simulink model "AGC_script"  (R2024b)
settings: Solver=VariableStepAuto  StartTime=0.0  StopTime=7*60  RelTol=1e-3
libraries: audiomeasurements x7, dspvision x7
settings Model: Creator=Pedro  LastModifiedBy=Pedro

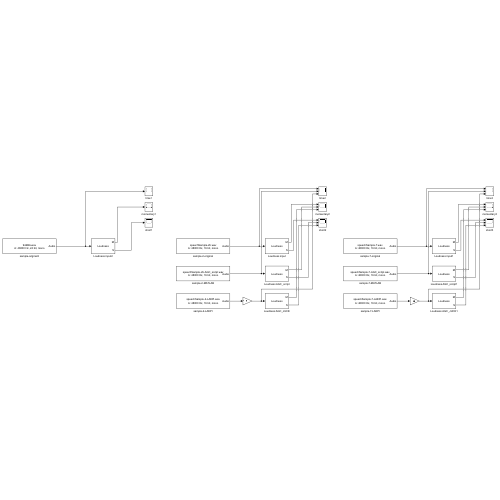
[thumbnail: Simulink's stored preview of the top-level diagram]
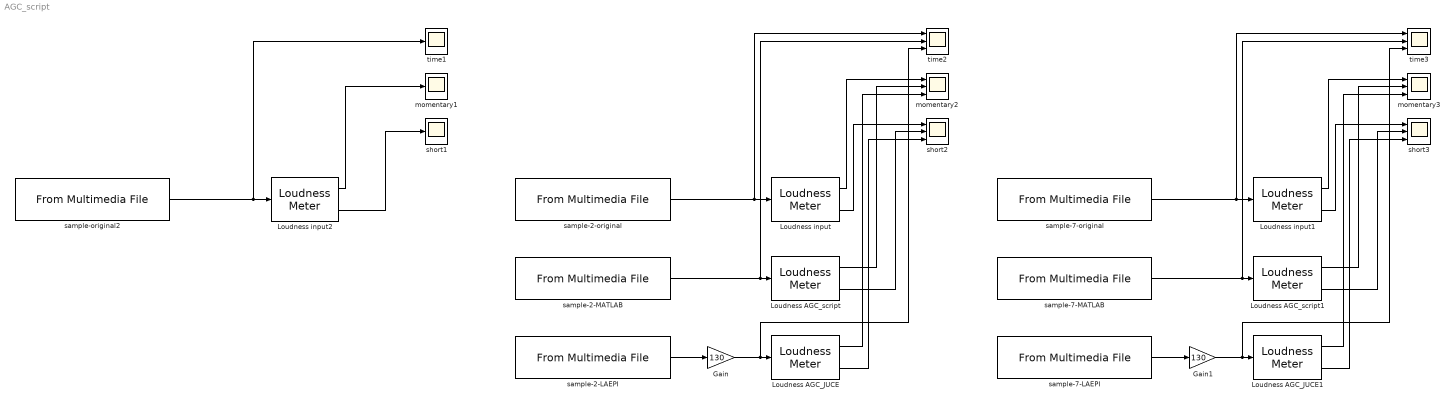
== system AGC_script ==
  Gain : Gain  Gain=130
  Gain1 : Gain  Gain=130
  Loudness AGC_JUCE : audiomeasurements/Loudness Meter  ChannelWeights=[ 1, 1, 1, 1.41, 1.41 ]  UseRelativeScale=off  TargetLoudness=-23.0  OutputTruePeak=off  InheritSampleRate=off  SampleRate=48000  SimulateUsing=Interpreted execution
  Loudness AGC_JUCE1 : audiomeasurements/Loudness Meter  ChannelWeights=[ 1, 1, 1, 1.41, 1.41 ]  UseRelativeScale=off  TargetLoudness=-23.0  OutputTruePeak=off  InheritSampleRate=off  SampleRate=48000  SimulateUsing=Interpreted execution
  Loudness AGC_script : audiomeasurements/Loudness Meter  ChannelWeights=[ 1, 1, 1, 1.41, 1.41 ]  UseRelativeScale=off  TargetLoudness=-23.0  OutputTruePeak=off  InheritSampleRate=off  SampleRate=48000  SimulateUsing=Interpreted execution
  Loudness AGC_script1 : audiomeasurements/Loudness Meter  ChannelWeights=[ 1, 1, 1, 1.41, 1.41 ]  UseRelativeScale=off  TargetLoudness=-23.0  OutputTruePeak=off  InheritSampleRate=off  SampleRate=48000  SimulateUsing=Interpreted execution
  Loudness input : audiomeasurements/Loudness Meter  ChannelWeights=[ 1, 1, 1, 1.41, 1.41 ]  UseRelativeScale=off  TargetLoudness=-23.0  OutputTruePeak=off  InheritSampleRate=off  SampleRate=48000  SimulateUsing=Interpreted execution
  Loudness input1 : audiomeasurements/Loudness Meter  ChannelWeights=[ 1, 1, 1, 1.41, 1.41 ]  UseRelativeScale=off  TargetLoudness=-23.0  OutputTruePeak=off  InheritSampleRate=off  SampleRate=48000  SimulateUsing=Interpreted execution
  Loudness input2 : audiomeasurements/Loudness Meter  ChannelWeights=[ 1, 1, 1, 1.41, 1.41 ]  UseRelativeScale=off  TargetLoudness=-23.0  OutputTruePeak=off  InheritSampleRate=off  SampleRate=48000  SimulateUsing=Interpreted execution
  momentary1 : Scope
  momentary2 : Scope  NumInputPorts=3
  momentary3 : Scope  NumInputPorts=3
  sample-2-LAEPI : dspvision/From Multimedia File  inputFilename=C:\Users\Pedro\My Drive\25.1\Projeto Integrador\MATLAB\teste-5\samples\speechSample-2-LAEPI.wav  readRange=[1 Inf]  loop=on  numPlays=1  outputStreams=Audio only  videoDataType=single  audioDataType=double  inheritSampleTime=on  userDefinedSampleTime=1/30  noAudioOutput=off  isIntensityVideo=off  fourcc=RGB  colorVideoFormat=Separate color signals  outputEOF=off  dataOrg=Column-major  audioFrameSize=1024  computeAudioFrameSize=off  outSamplingMode=Sample based
      settings: LibrarySourceBlock=audiosources/From Multimedia File
  sample-2-MATLAB : dspvision/From Multimedia File  inputFilename=C:\Users\Pedro\My Drive\25.1\Projeto Integrador\MATLAB\teste-5\samples\speechSample-2b-AGC_script.wav  readRange=[1 Inf]  loop=on  numPlays=1  outputStreams=Audio only  videoDataType=single  audioDataType=double  inheritSampleTime=on  userDefinedSampleTime=1/30  noAudioOutput=off  isIntensityVideo=off  fourcc=RGB  colorVideoFormat=Separate color signals  outputEOF=off  dataOrg=Column-major  audioFrameSize=1024  computeAudioFrameSize=off  outSamplingMode=Sample based
      settings: LibrarySourceBlock=audiosources/From Multimedia File
  sample-2-original : dspvision/From Multimedia File  inputFilename=C:\Users\Pedro\My Drive\25.1\Projeto Integrador\MATLAB\teste-5\samples\speechSample-2b.wav  readRange=[1 Inf]  loop=on  numPlays=1  outputStreams=Audio only  videoDataType=single  audioDataType=double  inheritSampleTime=on  userDefinedSampleTime=1/30  noAudioOutput=off  isIntensityVideo=off  fourcc=RGB  colorVideoFormat=Separate color signals  outputEOF=off  dataOrg=Column-major  audioFrameSize=1024  computeAudioFrameSize=off  outSamplingMode=Sample based
      settings: LibrarySourceBlock=audiosources/From Multimedia File
  sample-7-LAEPI : dspvision/From Multimedia File  inputFilename=C:\Users\Pedro\My Drive\25.1\Projeto Integrador\MATLAB\teste-5\samples\speechSample-7-LAEPI.wav  readRange=[1 Inf]  loop=on  numPlays=1  outputStreams=Audio only  videoDataType=single  audioDataType=double  inheritSampleTime=on  userDefinedSampleTime=1/30  noAudioOutput=off  isIntensityVideo=off  fourcc=RGB  colorVideoFormat=Separate color signals  outputEOF=off  dataOrg=Column-major  audioFrameSize=1024  computeAudioFrameSize=off  outSamplingMode=Sample based
      settings: LibrarySourceBlock=audiosources/From Multimedia File
  sample-7-MATLAB : dspvision/From Multimedia File  inputFilename=C:\Users\Pedro\My Drive\25.1\Projeto Integrador\MATLAB\teste-5\samples\speechSample-7-AGC_script.wav  readRange=[1 Inf]  loop=on  numPlays=1  outputStreams=Audio only  videoDataType=single  audioDataType=double  inheritSampleTime=on  userDefinedSampleTime=1/30  noAudioOutput=off  isIntensityVideo=off  fourcc=RGB  colorVideoFormat=Separate color signals  outputEOF=off  dataOrg=Column-major  audioFrameSize=1024  computeAudioFrameSize=off  outSamplingMode=Sample based
      settings: LibrarySourceBlock=audiosources/From Multimedia File
  sample-7-original : dspvision/From Multimedia File  inputFilename=C:\Users\Pedro\My Drive\25.1\Projeto Integrador\MATLAB\teste-5\samples\speechSample-7.wav  readRange=[1 Inf]  loop=on  numPlays=1  outputStreams=Audio only  videoDataType=single  audioDataType=double  inheritSampleTime=on  userDefinedSampleTime=1/30  noAudioOutput=off  isIntensityVideo=off  fourcc=RGB  colorVideoFormat=Separate color signals  outputEOF=off  dataOrg=Column-major  audioFrameSize=1024  computeAudioFrameSize=off  outSamplingMode=Sample based
      settings: LibrarySourceBlock=audiosources/From Multimedia File
  sample-original2 : dspvision/From Multimedia File  inputFilename=C:\Users\Pedro\My Drive\25.1\Projeto Integrador\MATLAB\teste-5\samples\94dBA.wav  readRange=[1 Inf]  loop=on  numPlays=inf  outputStreams=Audio only  videoDataType=single  audioDataType=double  inheritSampleTime=on  userDefinedSampleTime=1/30  noAudioOutput=off  isIntensityVideo=off  fourcc=RGB  colorVideoFormat=Separate color signals  outputEOF=off  dataOrg=Column-major  audioFrameSize=1024  computeAudioFrameSize=off  outSamplingMode=Sample based
      settings: LibrarySourceBlock=audiosources/From Multimedia File
  short1 : Scope
  short2 : Scope  NumInputPorts=3
  short3 : Scope  NumInputPorts=3
  time1 : Scope
  time2 : Scope  NumInputPorts=3
  time3 : Scope  NumInputPorts=3
  wires:
  sample-2-LAEPI/1 -> Gain/1
  sample-2-MATLAB/1 -> time2/2, Loudness AGC_script/1
  sample-2-original/1 -> time2/1, Loudness input/1
  Loudness AGC_JUCE/2 -> short2/3
  Loudness input/1 -> momentary2/1
  Loudness AGC_script/1 -> momentary2/2
  Loudness AGC_JUCE/1 -> momentary2/3
  Loudness input/2 -> short2/1
  Loudness AGC_script/2 -> short2/2
  Loudness AGC_script1/1 -> momentary3/2
  Loudness input1/2 -> short3/1
  Loudness AGC_JUCE1/2 -> short3/3
  Loudness AGC_script1/2 -> short3/2
  sample-7-MATLAB/1 -> time3/2, Loudness AGC_script1/1
  Loudness input1/1 -> momentary3/1
  sample-7-LAEPI/1 -> Gain1/1
  Loudness AGC_JUCE1/1 -> momentary3/3
  sample-7-original/1 -> time3/1, Loudness input1/1
  Loudness input2/2 -> short1/1
  Loudness input2/1 -> momentary1/1
  sample-original2/1 -> time1/1, Loudness input2/1
  Gain/1 -> time2/3, Loudness AGC_JUCE/1
  Gain1/1 -> time3/3, Loudness AGC_JUCE1/1
